simulink library "Lib_Piccolo"  (R2018b)
settings: Solver=VariableStepAuto  StartTime=0.0  StopTime=10.0  RelTol=1e-3
values from neighbouring files (symbols this model uses):
  AccelErrInt2Brakes = 0.15    [SimulationControlConfig16P.m]    (also in SimulationControlConfig16P_LEGACY.m; SimulationControlConfigTAILLESS.m = 0.2; SimulationControlConfigUTAIL.m = 0.2)
  AileronMax = 25    [SimulationControlConfig16P.m]    (also in SimulationControlConfig16P_LEGACY.m; SimulationControlConfigTAILLESS.m; SimulationControlConfigUTAIL.m)
  AileronPower = 0.00268    [SimulationControlConfig16P.m]    (also in SimulationControlConfig16P_LEGACY.m; SimulationControlConfigTAILLESS.m; SimulationControlConfigUTAIL.m)
  AileronSurfaceMax = 45    [SimulationControlConfig16P.m]    (also in SimulationControlConfig16P_LEGACY.m)
  AileronTrim = 0    [SimulationControlConfig16P.m]    (also in SimulationControlConfig16P_LEGACY.m; SimulationControlConfigTAILLESS.m; SimulationControlConfigUTAIL.m)
  Alt = 1000 + TerrainHeight    [SimulationStateConfig.m]
  AltCruise_m = testPlans(testIndx).terrainElevation * 0.3048 + 200    [SimulationControlConfig16P.m]    (also in SimulationControlConfigTAILLESS.m = 1083; SimulationControlConfigUTAIL.m = testPlans(testIndx).terrainElevation * 0.3048 + 152)
  AltitudeRate2PitchCmdIntegratorInit = 0.1    [SimulationControlPre.m]
  AltMax = 10000    [SimulationControlConfig16P.m]    (also in SimulationControlConfig16P_LEGACY.m; SimulationControlConfigTAILLESS.m; SimulationControlConfigUTAIL.m)
  AltMaxAccel = 1.25    [SimulationControlConfig16P.m]    (also in SimulationControlConfig16P_LEGACY.m = 0.9; SimulationControlConfigTAILLESS.m = 1.7; SimulationControlConfigUTAIL.m = 2)
  AltMin = 0    [SimulationControlConfig16P.m]    (also in SimulationControlConfig16P_LEGACY.m; SimulationControlConfigTAILLESS.m; SimulationControlConfigUTAIL.m)
  AltRateCmd2Pitch = 0.50    (= 0.5)    [SimulationControlConfig16P.m]    (also in SimulationControlConfig16P_LEGACY.m = 0.6; SimulationControlConfigTAILLESS.m = 0.2; SimulationControlConfigUTAIL.m = 0.3)
  AltRateError2Pitch = 0.40    (= 0.4)    [SimulationControlConfig16P.m]    (also in SimulationControlConfig16P_LEGACY.m; SimulationControlConfigTAILLESS.m = 0.55; SimulationControlConfigUTAIL.m = 0.55)
  AltRateErrorInt2Pitch = 0.50    (= 0.5)    [SimulationControlConfig16P.m]    (also in SimulationControlConfig16P_LEGACY.m = 0.45; SimulationControlConfigTAILLESS.m; SimulationControlConfigUTAIL.m = 0.75)
  AltRateLpfCutOff = 3    [SimulationControlConfig16P.m]    (also in SimulationControlConfig16P_LEGACY.m; SimulationControlConfigTAILLESS.m = 2; SimulationControlConfigUTAIL.m = 2)
  AutoNosegear2Rudder = 26    [SimulationControlConfig16P.m]    (also in SimulationControlConfig16P_LEGACY.m; SimulationControlConfigTAILLESS.m = 25.2; SimulationControlConfigUTAIL.m = 14)
  b = 5.54    [SimulationControlConfig16P.m]    (also in SimulationControlConfig16P_LEGACY.m; SimulationControlConfigTAILLESS.m = 2.37; SimulationControlConfigUTAIL.m = 2.37)
  Bank2AileronIntegratorInit = 0    [SimulationControlPre.m]
  BankMax_User = BankMax_User/180*pi    (= 0.523598775598)    [SimulationControlConfig16P.m]    (also in SimulationControlConfig16P_LEGACY.m; SimulationControlConfigTAILLESS.m = 0.610865238198; SimulationControlConfigUTAIL.m = 0.628318530718)
  baseLegFlaps = 20    [SimulationControlConfig16P.m]    (also in SimulationControlConfig16P_LEGACY.m = 0; SimulationControlConfigTAILLESS.m = 15; SimulationControlConfigUTAIL.m = 10)
  C = GeneticOpt.C    [SimulationCostFunction.m]
  c = Sw/b    (= 0.841696750903)    [SimulationControlConfig16P.m]    (also in SimulationControlConfig16P_LEGACY.m; SimulationControlConfigTAILLESS.m = 0.354008438819; SimulationControlConfigUTAIL.m = 0.354008438819)
  cell2WheelFactorMG = 5.98    [SimulationSensorConfig16P_LEGACY.m]
  cell2WheelFactorNG = 1    [SimulationSensorConfig16P_LEGACY.m]
  cellSatMaxMG = 15000    [SimulationSensorConfig16P.m]    (also in SimulationSensorConfig16P_LEGACY.m; SimulationSensorConfigTAILLESS7P.m; SimulationSensorConfigUTAIL7P.m)
  cellSatMaxNG = 1000    [SimulationSensorConfig16P.m]    (also in SimulationSensorConfig16P_LEGACY.m; SimulationSensorConfigTAILLESS7P.m; SimulationSensorConfigUTAIL7P.m)
  cellSatMinMG = -15000    [SimulationSensorConfig16P.m]    (also in SimulationSensorConfig16P_LEGACY.m; SimulationSensorConfigTAILLESS7P.m; SimulationSensorConfigUTAIL7P.m)
  cellSatMinNG = -1000    [SimulationSensorConfig16P.m]    (also in SimulationSensorConfig16P_LEGACY.m; SimulationSensorConfigTAILLESS7P.m; SimulationSensorConfigUTAIL7P.m)
  CL_Limit = CL_Max    (= 0.54)    [SimulationControlConfig16P.m]    (also in SimulationControlConfig16P_LEGACY.m; SimulationControlConfigTAILLESS.m; SimulationControlConfigUTAIL.m = 0.53)
  CL_Max = 0.54    [SimulationControlConfig16P.m]    (also in SimulationControlConfig16P_LEGACY.m; SimulationControlConfigTAILLESS.m; SimulationControlConfigUTAIL.m = 0.53)
  CL_Max_Nom = 0.465    [SimulationControlConfig16P.m]    (also in SimulationControlConfig16P_LEGACY.m; SimulationControlConfigTAILLESS.m = 0.39; SimulationControlConfigUTAIL.m)
  CL_Min = 0    [SimulationControlConfig16P.m]    (also in SimulationControlConfig16P_LEGACY.m; SimulationControlConfigTAILLESS.m; SimulationControlConfigUTAIL.m)
  ClimbMaxFraction = 0.35    [SimulationControlConfig16P.m]    (also in SimulationControlConfig16P_LEGACY.m = 0.24; SimulationControlConfigTAILLESS.m = 0.19; SimulationControlConfigUTAIL.m = 0.21)
  ClimboutMaxBank = 7.0    (= 7)    [SimulationControlConfig16P.m]    (also in SimulationControlConfig16P_LEGACY.m; SimulationControlConfigTAILLESS.m = 5; SimulationControlConfigUTAIL.m)
  ClimboutTimer = 7.0    (= 7)    [SimulationControlConfig16P.m]    (also in SimulationControlConfig16P_LEGACY.m; SimulationControlConfigTAILLESS.m; SimulationControlConfigUTAIL.m)
  dCl_per_dFlap = 0.005581818    [SimulationControlConfig16P.m]    (also in SimulationControlConfig16P_LEGACY.m = 0; SimulationControlConfigTAILLESS.m = 0; SimulationControlConfigUTAIL.m = 0)
  DecelerationCmd = 3.1    [SimulationControlConfig16P.m]    (also in SimulationControlConfig16P_LEGACY.m; SimulationControlConfigTAILLESS.m = 0.1; SimulationControlConfigUTAIL.m = 0.1)
  DeRotateLogicEndTimer = abs((NoseDownLimit_Deg-1)/DeRotateRamp_Dps)    [SimulationControlConfig16P.m]    (also in SimulationControlConfig16P_LEGACY.m; SimulationControlConfigTAILLESS.m; SimulationControlConfigUTAIL.m)
  DeRotateLogicHoldNoseUpTimer = 0.1    [SimulationControlConfig16P.m]    (also in SimulationControlConfig16P_LEGACY.m; SimulationControlConfigTAILLESS.m; SimulationControlConfigUTAIL.m)
  DeRotateLogicTimerTimeout = 2    [SimulationControlConfig16P.m]    (also in SimulationControlConfig16P_LEGACY.m; SimulationControlConfigTAILLESS.m; SimulationControlConfigUTAIL.m)
  DeRotateLowerCmdSaturation = 0    [SimulationControlConfig16P.m]    (also in SimulationControlConfig16P_LEGACY.m; SimulationControlConfigTAILLESS.m; SimulationControlConfigUTAIL.m)
  DeRotateRamp_Dps = 3    [SimulationControlConfig16P.m]    (also in SimulationControlConfig16P_LEGACY.m; SimulationControlConfigTAILLESS.m = 8; SimulationControlConfigUTAIL.m = 8)
  DeRotateUpperCmdSaturation = 7    [SimulationControlConfig16P.m]    (also in SimulationControlConfig16P_LEGACY.m; SimulationControlConfigTAILLESS.m; SimulationControlConfigUTAIL.m)
  DescentMaxFraction = 0.22    [SimulationControlConfig16P.m]    (also in SimulationControlConfig16P_LEGACY.m = 0.2; SimulationControlConfigTAILLESS.m = 0.17; SimulationControlConfigUTAIL.m = 0.17)
  DesktopSimTerrainOffset_m = 0.406    [SimulationAircraftConfig.m]
  downwindFlaps = 0    [SimulationControlConfig16P.m]    (also in SimulationControlConfig16P_LEGACY.m; SimulationControlConfigTAILLESS.m; SimulationControlConfigUTAIL.m)
  DP_init = 0.5*1.225*V_init^2    [SimulationControlConfig16P.m]    (also in SimulationControlConfig16P_LEGACY.m; SimulationControlConfigTAILLESS.m; SimulationControlConfigUTAIL.m)
  dscNoiseMG = 1    [SimulationSensorConfig16P_LEGACY.m]
  dscNoiseNG = 0.25    [SimulationSensorConfig16P_LEGACY.m]
  DSCnumBits = 24    [SimulationSensorConfig16P.m]    (also in SimulationSensorConfig16P_LEGACY.m; SimulationSensorConfigTAILLESS7P.m; SimulationSensorConfigUTAIL7P.m)
  DSCRangeMaxMG = 15000    [SimulationSensorConfig16P.m]    (also in SimulationSensorConfig16P_LEGACY.m; SimulationSensorConfigTAILLESS7P.m; SimulationSensorConfigUTAIL7P.m)
  DSCRangeMaxNG = 1000    [SimulationSensorConfig16P.m]    (also in SimulationSensorConfig16P_LEGACY.m; SimulationSensorConfigTAILLESS7P.m; SimulationSensorConfigUTAIL7P.m)
  DSCRangeMinMG = -15000    [SimulationSensorConfig16P.m]    (also in SimulationSensorConfig16P_LEGACY.m; SimulationSensorConfigTAILLESS7P.m; SimulationSensorConfigUTAIL7P.m)
  DSCRangeMinNG = -1000    [SimulationSensorConfig16P.m]    (also in SimulationSensorConfig16P_LEGACY.m; SimulationSensorConfigTAILLESS7P.m; SimulationSensorConfigUTAIL7P.m)
  dt = DLLSim.dt    [SimulationTimeStep.m]    (also in SimulationTrim.m = 0.02)
  EarlyTouchdownThreshold = 3.0    (= 3)    [SimulationControlConfig16P.m]    (also in SimulationControlConfig16P_LEGACY.m; SimulationControlConfigTAILLESS.m = 2.2; SimulationControlConfigUTAIL.m = 2.5)
  ElevatorDeflectionRate = 15    [SimulationControlConfig16P.m]    (also in SimulationControlConfig16P_LEGACY.m = 12; SimulationControlConfigTAILLESS.m = 10; SimulationControlConfigUTAIL.m = 12)
  ElevatorMax = 25    [SimulationControlConfig16P.m]    (also in SimulationControlConfig16P_LEGACY.m; SimulationControlConfigTAILLESS.m; SimulationControlConfigUTAIL.m)
  ElevatorPower = -0.002209    [SimulationControlConfig16P.m]    (also in SimulationControlConfig16P_LEGACY.m; SimulationControlConfigTAILLESS.m = -0.002956; SimulationControlConfigUTAIL.m = -0.00205983)
  ElevatorTrim = -3.5    [SimulationControlConfig16P.m]    (also in SimulationControlConfig16P_LEGACY.m; SimulationControlConfigTAILLESS.m = -6; SimulationControlConfigUTAIL.m = -8)
  elevonBias = 0    [SimulationControlConfig16P.m]    (also in SimulationControlConfig16P_LEGACY.m; SimulationControlConfigTAILLESS.m; SimulationControlConfigUTAIL.m)
  Enable_TAS_Protection = 0    [SimulationControlConfig16P.m]    (also in SimulationControlConfig16P_LEGACY.m; SimulationControlConfigTAILLESS.m; SimulationControlConfigUTAIL.m)
  EnableCrossTrackAbort = 1    [SimulationControlConfig16P.m]    (also in SimulationControlConfigTAILLESS.m; SimulationControlConfigUTAIL.m)
  EnergyBandwidth = 0.02    [SimulationControlConfig16P.m]    (also in SimulationControlConfig16P_LEGACY.m; SimulationControlConfigTAILLESS.m = 0.06; SimulationControlConfigUTAIL.m = 0.06)
  EngineLhFuelCut = 0    [SimulationAircraftConfig.m]
  EngineRhFuelCut = 0    [SimulationAircraftConfig.m]
  FastThrottleRate = 0.075    [SimulationControlConfig16P.m]    (also in SimulationControlConfig16P_LEGACY.m = 0.05; SimulationControlConfigTAILLESS.m = 0.1; SimulationControlConfigUTAIL.m = 0.1)
  FilterWarmUpTime = 2    [SimulationSensorConfig16P.m]    (also in SimulationSensorConfig16P_LEGACY.m; SimulationSensorConfigTAILLESS7P.m; SimulationSensorConfigUTAIL7P.m)
  finalApproachFlaps = 20    [SimulationControlConfig16P.m]    (also in SimulationControlConfig16P_LEGACY.m = 0; SimulationControlConfigTAILLESS.m = 22; SimulationControlConfigUTAIL.m = 10)
  FinalDescentSlope_Deg = testPlans(testIndx).descentSlope    [SimulationControlConfig16P.m]    (also in SimulationControlConfig16P_LEGACY.m; SimulationControlConfigTAILLESS.m; SimulationControlConfigUTAIL.m)
  flapMax = 0    [SimulationControlConfig16P.m]    (also in SimulationControlConfig16P_LEGACY.m; SimulationControlConfigTAILLESS.m; SimulationControlConfigUTAIL.m)
  flapRate = 7.5    [SimulationControlConfig16P.m]    (also in SimulationControlConfig16P_LEGACY.m; SimulationControlConfigTAILLESS.m = 6.6; SimulationControlConfigUTAIL.m)
  FlareHeight = 5    [SimulationControlConfig16P.m]    (also in SimulationControlConfig16P_LEGACY.m = 4.8; SimulationControlConfigTAILLESS.m = 2.5; SimulationControlConfigUTAIL.m = 2)
  FlareVerticalRate_mps = -0.4    [SimulationControlConfig16P.m]    (also in SimulationControlConfig16P_LEGACY.m = -0.5; SimulationControlConfigTAILLESS.m = -0.15; SimulationControlConfigUTAIL.m = -0.15)
  Fp_Aileron = 0.55*2*pi*RollRateLpfCutoff*dt    [SimulationControlConfig16P.m]    (also in SimulationControlConfig16P_LEGACY.m; SimulationControlConfigTAILLESS.m; SimulationControlConfigUTAIL.m)
  Fp_Alt = 0.55*AltBandwidth    (= 0.099)    [SimulationControlConfig16P.m]    (also in SimulationControlConfig16P_LEGACY.m; SimulationControlConfigTAILLESS.m = 0.587477826221; SimulationControlConfigUTAIL.m = 0.69115038379)
  Fp_AltRate = 0.55*2*pi*AltRateLpfCutOff*dt    [SimulationControlConfig16P.m]    (also in SimulationControlConfig16P_LEGACY.m; SimulationControlConfigTAILLESS.m; SimulationControlConfigUTAIL.m)
  Fp_Elevator = 0.55*2*pi*PitchRateLpfCutoff*dt    [SimulationControlConfig16P.m]    (also in SimulationControlConfig16P_LEGACY.m; SimulationControlConfigTAILLESS.m; SimulationControlConfigUTAIL.m)
  Fp_Energy = 0.55*2*pi*EnergyBandwidth    (= 0.069115038379)    [SimulationControlConfig16P.m]    (also in SimulationControlConfig16P_LEGACY.m; SimulationControlConfigTAILLESS.m = 0.207345115137; SimulationControlConfigUTAIL.m = 0.207345115137)
  Fp_Energy2 = 0.55*2*pi*EnergyBandwidth*dt    [SimulationControlConfig16P.m]    (also in SimulationControlConfig16P_LEGACY.m; SimulationControlConfigTAILLESS.m; SimulationControlConfigUTAIL.m)
  Fp_Pitch = 0.55*2*pi*PitchBandwidth    (= 2.76460153516)    [SimulationControlConfig16P.m]    (also in SimulationControlConfig16P_LEGACY.m = 3.11017672705; SimulationControlConfigTAILLESS.m = 3.80132711084; SimulationControlConfigUTAIL.m = 2.41902634326)
  Fp_Pitch_2 = 0.55*2*pi*PitchBandwidth*dt    [SimulationControlConfig16P.m]    (also in SimulationControlConfig16P_LEGACY.m; SimulationControlConfigTAILLESS.m; SimulationControlConfigUTAIL.m)
  Fp_Roll = RollBandwidth^2    (= 1)    [SimulationControlConfig16P.m]    (also in SimulationControlConfig16P_LEGACY.m = 1.44; SimulationControlConfigTAILLESS.m; SimulationControlConfigUTAIL.m)
  Fp_Rudder = 0.55*2*pi*YawRateLpfCutoff*dt    [SimulationControlConfig16P.m]    (also in SimulationControlConfig16P_LEGACY.m; SimulationControlConfigTAILLESS.m; SimulationControlConfigUTAIL.m)
  Fp_TAS = 0.55*2*pi*TASBandwidth    (= 0.103672557568)    [SimulationControlConfig16P.m]    (also in SimulationControlConfig16P_LEGACY.m; SimulationControlConfigTAILLESS.m = 0.172787595947; SimulationControlConfigUTAIL.m = 0.172787595947)
  Fp_TAS_Filter = 2*pi*TasLpfCutoff*dt    [SimulationControlConfig16P.m]    (also in SimulationControlConfig16P_LEGACY.m; SimulationControlConfigTAILLESS.m; SimulationControlConfigUTAIL.m)
  Fp_Turn = 0.55*2*pi*TurnErrLPFcutoff    (= 0.0345575191895)    [SimulationControlConfig16P.m]    (also in SimulationControlConfig16P_LEGACY.m; SimulationControlConfigTAILLESS.m = 0.172787595947; SimulationControlConfigUTAIL.m = 0.172787595947)
  Fp_TurnDerr = 0.55*2*pi*TurnDerivativeLPFcutoff    (= 0.0345575191895)    [SimulationControlConfig16P.m]    (also in SimulationControlConfig16P_LEGACY.m; SimulationControlConfigTAILLESS.m = 0.172787595947; SimulationControlConfigUTAIL.m = 0.172787595947)
  FTV = 3    [SimulationAircraftConfig.m]
  ftvStaticPositionError = 1/1.18    (= 0.847457627119)    [SimulationSensorConfig16P.m]    (also in SimulationSensorConfig16P_LEGACY.m; SimulationSensorConfigTAILLESS7P.m = 1; SimulationSensorConfigUTAIL7P.m = 1)
  g = 9.81    [SimulationStateConfig.m]
  GustSpd_Kts = testPlans(testIndx).gustSpd    [SimulationStateConfig.m]
  GustTriggerVal = testPlans(testIndx).gustTriggerVal    [SimulationStateConfig.m]
  HeadingErr2TurnRate = 0.5    [SimulationControlConfig16P.m]    (also in SimulationControlConfig16P_LEGACY.m; SimulationControlConfigTAILLESS.m; SimulationControlConfigUTAIL.m)
  HeadingErrDer2TurnRate = 0.3    [SimulationControlConfig16P.m]    (also in SimulationControlConfig16P_LEGACY.m; SimulationControlConfigTAILLESS.m; SimulationControlConfigUTAIL.m)
  IASbounce = IASstall*0.8    [SimulationControlPre.m]
  IAScruiseCMD = sqrt(2*m*9.81/(1.225*Sw*CL_cruise))    [SimulationControlConfig16P.m]    (also in SimulationControlConfig16P_LEGACY.m; SimulationControlConfigTAILLESS.m; SimulationControlConfigUTAIL.m)
  IASfinalCMD = 1.12 * IASmin    [SimulationControlConfig16P.m]    (also in SimulationControlConfig16P_LEGACY.m = 1.10 * IASmin; SimulationControlConfigTAILLESS.m = 1.10 * IASmin; SimulationControlConfigUTAIL.m = 1.15 * IASmin)
  IASflareCMD = IASstall    [SimulationControlConfig16P.m]    (also in SimulationControlConfig16P_LEGACY.m; SimulationControlConfigTAILLESS.m; SimulationControlConfigUTAIL.m)
  IASmax = 64    [SimulationControlConfig16P.m]    (also in SimulationControlConfig16P_LEGACY.m = 46; SimulationControlConfigTAILLESS.m = 38.58; SimulationControlConfigUTAIL.m = 35)
  IASmin = sqrt(2*m*9.81/(1.225*Sw*0.9*CL_Max_Nom))    [SimulationControlConfig16P.m]    (also in SimulationControlConfig16P_LEGACY.m; SimulationControlConfigTAILLESS.m; SimulationControlConfigUTAIL.m)
  IASshortCMD = IASstall    [SimulationControlConfig16P.m]    (also in SimulationControlConfig16P_LEGACY.m; SimulationControlConfigTAILLESS.m; SimulationControlConfigUTAIL.m)
  IASstall = sqrt(2*m*9.81/(1.225*Sw*CL_Max))    [SimulationControlConfig16P.m]    (also in SimulationControlConfig16P_LEGACY.m; SimulationControlConfigTAILLESS.m; SimulationControlConfigUTAIL.m)
  inFlight = 1    [SimulationControlConfig16P.m]    (also in SimulationControlConfigTAILLESS.m; SimulationControlConfigUTAIL.m)
  JetCatOffset = 5    [SimulationControlConfig16P.m]    (also in SimulationControlConfig16P_LEGACY.m)
  LaunchRollingElevator = -1.5    [SimulationControlConfig16P.m]    (also in SimulationControlConfig16P_LEGACY.m; SimulationControlConfigTAILLESS.m = 1; SimulationControlConfigUTAIL.m = 1)
  ldg_NosegearMax = 10    [SimulationControlConfig16P.m]    (also in SimulationControlConfig16P_LEGACY.m; SimulationControlConfigTAILLESS.m; SimulationControlConfigUTAIL.m)
  ldg_TrackVyErrInt2Nosegear = 0.1250    (= 0.125)    [SimulationControlConfig16P.m]    (also in SimulationControlConfig16P_LEGACY.m; SimulationControlConfigTAILLESS.m = 0.00714285714286; SimulationControlConfigUTAIL.m = 0.00714285714286)
  ldg_TrackVyErrPro2Nosegear = 0.35    [SimulationControlConfig16P.m]    (also in SimulationControlConfig16P_LEGACY.m; SimulationControlConfigTAILLESS.m = 0.0546666666667; SimulationControlConfigUTAIL.m = 0.0546666666667)
  ldg_TrackY2Vy = 0.07    [SimulationControlConfig16P.m]    (also in SimulationControlConfig16P_LEGACY.m; SimulationControlConfigTAILLESS.m = 0.17; SimulationControlConfigUTAIL.m = 0.17)
  ldg_Vy2NosegearScalingPower = 1.075    [SimulationControlConfig16P.m]    (also in SimulationControlConfig16P_LEGACY.m; SimulationControlConfigTAILLESS.m = 0.6; SimulationControlConfigUTAIL.m = 0.5)
  ldg_Y2VyScalingPower = 0.175    [SimulationControlConfig16P.m]    (also in SimulationControlConfig16P_LEGACY.m; SimulationControlConfigTAILLESS.m = 0; SimulationControlConfigUTAIL.m = 0)
  ldg_YawRate2Nosegear = 0.175    [SimulationControlConfig16P.m]    (also in SimulationControlConfig16P_LEGACY.m; SimulationControlConfigTAILLESS.m = 0.065; SimulationControlConfigUTAIL.m = 0.065)
  LiftSlope = 0.064285    [SimulationControlConfig16P.m]    (also in SimulationControlConfig16P_LEGACY.m; SimulationControlConfigTAILLESS.m = 0.058631; SimulationControlConfigUTAIL.m)
  LPFaileronInit = 0    [SimulationControlPre.m]
  LPFclestInit = 0    [SimulationControlPre.m]
  LPFenergyFFInit = 0    [SimulationControlPre.m]
  LPFtasInit = V_init + 2    [SimulationControlPre.m]
  LPFthrottleInit = ThrottleTrim    [SimulationControlPre.m]
  LPFturnErrInit = 0    [SimulationControlPre.m]
  ... (+115 more)
undefined symbols (not defined in the file or in its folder): abortFlag, alphaHPF, apmDelay, BRWNOUT, CRAWOR, CRAWUR, DiscIntNeverNeededParam, DLLSim, DLLSimStep, ECOMOR, ECOMUR, Fp_Tas, GustTrigger_HeightAgl_m, IPSTAT, LCINTEG, Ldg_Persist_Time, LOWER_FLAGS, MSG_ENABLE, NoiseStd, OLDVAL, OVERRIDE_ENABLE, OVERRIDE_VALUE, REBOOT, reversionEnable, revIASMax, revIASMin, revPitchMax, revPitchMin, revPitchRateMax, revRollMax, revRollRateMax, SAMPLE, SCALON, SensorModel, sigbuilder_block, Sim_Vx, Sim_Vy, Sim_Vz, Sim_Xpos, Sim_Ypos, Sim_Zpos, SYSOR, SYSUR, TARE, TEMPOR, TEMPUR, testIndx, testPlan, testPlans, Trim_piccoloInCmd, Trim_REFSI_FD_IN_nmodeCgShifterCmd_Ft, Trim_REFSI_FD_IN_nmodeFlapLhIBCmd_Deg, Trim_REFSI_FD_IN_nmodeFlapLhOBCmd_Deg, Trim_REFSI_FD_IN_nmodeFlapRhIBCmd_Deg, Trim_REFSI_FD_IN_nmodeFlapRhOBCmd_Deg, Trim_REFSI_FD_IN_nmodeSlatLhCmd_Deg, Trim_REFSI_FD_IN_nmodeSlatRhCmd_Deg, Trim_REFSI_FD_IN_nmodeSplrLhInbdCmd_Deg, Trim_REFSI_FD_IN_nmodeSplrLhOutbdCmd_Deg ... (+5)
libraries: simulink x866, aerolibconvert2 x60, $bdroot x52, aerolibatmos2 x5, dspswit3 x5, simulink_extras x4, dsparch4 x2, Lib_Piccolo_Alt x2, eeGeneralControl x1, dspindex x1
(part 10 of 44)

== system Lib_Piccolo/Control Allocation/M2 ==
  note: For 16.5% U-tail:
      | Aileron: aileron, inboard elevon, outboard elevon
      | Elevator: aft-flap, U-tail elevator,
      | Rudder: pylon rudder, winglet rudder, U-tail rudder
      |
      | For 16.5% Tailless (w/o U-tail elevator and U-tail rudder):
      | Aileron: aileron, inboard elevon, outboard elevon
      | Elevator: aft-flap, inboard elvon, outboard elevon
      | Rudder: pylon rudder, winglet rudder
  Aileron : Inport
  Elevator : Inport  Port=2
  Rudder : Inport  Port=3
  Throttle : Inport  Port=4
  Nosegear : Inport  Port=5
  Brake : Inport  Port=6
  Flap : Inport  Port=7
  Feedback Bus : Inport  Port=8
  Bus Creator : BusCreator  Inputs=10
  Bus Creator1 : BusCreator  Inputs=4
  Bus Creator2 : BusCreator  Inputs=2
  Bus Creator3 : BusCreator  Inputs=2
  Bus Creator4 : BusCreator  Inputs=2
  Constant : Constant  Value=FTV
  Constant1 : Constant  Value=0
  Constant2 : Constant  Value=elevonBias
  Gain{1..5,8..9,12,14,16..17} (11 alike) : Gain
  Gain{10..11,13,15} (4 alike) : Gain  Gain=-1
  Signal Specification : SignalSpecification  Dimensions=[1 1]  SampleTime=dt
  Signal Specification1 : SignalSpecification  Dimensions=[1 1]  SampleTime=dt
  Signal Specification2 : SignalSpecification  Dimensions=[1 1]  SampleTime=dt
  SlatLhPosnDeg : Constant  Value=Trim_REFSI_FD_IN_nmodeSlatLhCmd_Deg
  StabCmdDeg : Constant  Value=Trim_REFSI_FD_IN_nmodeStabCmd
  Surface Mixing Function : MATLAB Function  TreatAsAtomicUnit=on
  Switch : Switch  Criteria=u2 > Threshold  Threshold=2
  Terminator : Terminator
  Variant Model : $bdroot/Control Allocation/M2 Flap-to-Drag /Variant Model  SystemSampleTime=-1
  nmodeTlaLhCmdDeg3 : Constant  Value=Trim_REFSI_FD_IN_nmodeSplrLhOutbdCmd_Deg
  "Aileron_Deg " : Outport
  "InboardElevon_Deg " : Outport  Port=2
  OutboardElevon_Deg : Outport  Port=3
  "U-TailElevator_Deg " : Outport  Port=4
  Aft-Flap_Deg : Outport  Port=5
  PylonRudder_Deg : Outport  Port=6
  WingletRudder_Deg : Outport  Port=7
  U-tailRudder_Deg : Outport  Port=8
  "Throttle_Pct " : Outport  Port=9
  Nosegear_Deg : Outport  Port=10
  Brake (0-1) : Outport  Port=11
  Flaps_Deg : Outport  Port=12
  Slats_Deg : Outport  Port=13
  Spoilers_Deg : Outport  Port=14
  Stabilizer_Deg : Outport  Port=15
  tag scope: Sim_Surface=global
  wires:
  Elevator/1 -> Bus Creator/2, Signal Specification1/1  "Sim_ElevatorCmd"
  Aileron/1 -> Bus Creator/1, Signal Specification/1  "Sim_AileronCmd"
  Rudder/1 -> Bus Creator/3, Signal Specification2/1  "Sim_RudderCmd"
  Nosegear/1 -> Bus Creator/5, Nosegear_Deg/1  "Sim_NosegearCmd"
  Brake/1 -> Brake (0-1)/1, Bus Creator/6  "Sim_BrakeCmd"
  Bus Creator/1 -> [Sim_Surface]
  Throttle/1 -> Variant Model/1, Bus Creator/4  "Sim_ThrottleCmd"
  Variant Model/1 -> Gain16/1, Gain17/1  "Sim_ThrottleCmd"
  Bus Creator1/1 -> "Aileron_Deg "/1
  Bus Creator2/1 -> "InboardElevon_Deg "/1
  Bus Creator3/1 -> OutboardElevon_Deg/1
  Gain8/1 -> Bus Creator1/1  "PrtAileronUpperCmd_Deg"
  Gain9/1 -> Bus Creator1/2  "PrtAileronLowerCmd_Deg"
  Gain10/1 -> Bus Creator1/3  "StbdAileronUpperCmd_Deg"
  Gain11/1 -> Bus Creator1/4  "StbdAileronLowerCmd_Deg"
  Gain12/1 -> Bus Creator2/1  "PrtInbElevonCmd_Deg"
  Gain13/1 -> Bus Creator2/2  "StbdInbElevonCmd_Deg"
  Gain14/1 -> Bus Creator3/1  "PrtOutElevonCmd_Deg"
  Gain15/1 -> Bus Creator3/2  "StbdOutElevonCmd_Deg"
  Gain16/1 -> Bus Creator4/1  "PrtThrottleCmd_Pct"
  Bus Creator4/1 -> "Throttle_Pct "/1
  Gain17/1 -> Bus Creator4/2  "StbdThrottleCmd_Pct"
  SlatLhPosnDeg/1 -> Bus Creator/8, Slats_Deg/1  "Sim_SlatsCmd"
  nmodeTlaLhCmdDeg3/1 -> Bus Creator/9, Spoilers_Deg/1  "Sim_SpoilersCmd"
  Feedback Bus/1 -> Terminator/1
  StabCmdDeg/1 -> Bus Creator/10, Stabilizer_Deg/1  "Sim_StabilizerCmd"
  Flap/1 -> Surface Mixing Function/4(Pic_FlapCmd), Bus Creator/7, Flaps_Deg/1  "Sim_FlapsCmd"
  Surface Mixing Function/1(PrtAileronUpperCmd) -> Gain8/1
  Surface Mixing Function/2(PrtAileronLowerCmd) -> Gain9/1
  Surface Mixing Function/3(StbdAileronUpperCmd) -> Gain10/1
  Surface Mixing Function/4(StbdAileronLowerCmd) -> Gain11/1
  Surface Mixing Function/13(UTailRudderCmd) -> Gain5/1
  Surface Mixing Function/12(WingletRudderCmd) -> Gain4/1
  Surface Mixing Function/11(PylonRudderCmd) -> Gain3/1
  Surface Mixing Function/10(AftFlapCmd) -> Gain2/1
  Surface Mixing Function/9(ElevatorUtailCmd) -> Gain1/1
  Surface Mixing Function/8(StbdOutdElevonCmd) -> Gain15/1
  Surface Mixing Function/7(PrtOutElevonCmd) -> Gain14/1
  Surface Mixing Function/6(StbdInbdElevonCmd) -> Gain13/1
  Surface Mixing Function/5(PrtInbElevonCmd) -> Gain12/1
  Gain1/1 -> "U-TailElevator_Deg "/1  "UtailElevator_Deg"
  Gain2/1 -> Aft-Flap_Deg/1  "AftFlap_deg"
  Gain3/1 -> PylonRudder_Deg/1  "PylonRudder_Deg"
  Gain5/1 -> U-tailRudder_Deg/1  "UtailRudder_Deg"
  Signal Specification/1 -> Surface Mixing Function/1(Pic_AileronCmd)
  Signal Specification2/1 -> Surface Mixing Function/3(Pic_RudderCmd)
  Signal Specification1/1 -> Surface Mixing Function/2(Pic_ElevatorCmd)
  Constant/1 -> Switch/2
  Switch/1 -> WingletRudder_Deg/1  "WingletRudder_Deg"
  Constant1/1 -> Switch/3
  Gain4/1 -> Switch/1
  Constant2/1 -> Surface Mixing Function/5(elevonBias)

== system Lib_Piccolo/Control Allocation/M2 Flap-to-Drag  ==
  note: For 16.5% U-tail:
      | Aileron: aileron, inboard elevon, outboard elevon
      | Elevator: aft-flap, U-tail elevator,
      | Rudder: pylon rudder, winglet rudder, U-tail rudder
      |
      | For 16.5% Tailless (w/o U-tail elevator and U-tail rudder):
      | Aileron: aileron, inboard elevon, outboard elevon
      | Elevator: aft-flap, inboard elvon, outboard elevon
      | Rudder: pylon rudder, winglet rudder
  Aileron : Inport
  Elevator : Inport  Port=2
  Rudder : Inport  Port=3
  Throttle : Inport  Port=4
  Nosegear : Inport  Port=5
  Brake : Inport  Port=6
  Flap : Inport  Port=7
  Feedback Bus : Inport  Port=8
  Bus Creator : BusCreator  Inputs=10
  Bus Creator1 : BusCreator  Inputs=4
  Bus Creator2 : BusCreator  Inputs=2
  Bus Creator3 : BusCreator  Inputs=2
  Bus Creator4 : BusCreator  Inputs=2
  Constant : Constant  Value=FTV
  Constant1 : Constant  Value=0
  Constant2 : Constant  Value=elevonBias
  Constant3 : Constant  Value=AileronSurfaceMax
  FlapLhIBCmdDeg : Constant  Commented=on  Value=Trim_REFSI_FD_IN_nmodeFlapLhIBCmd_Deg
  FlapLhIBCmdDeg1 : Constant  Value=Trim_REFSI_FD_IN_nmodeFlapLhIBCmd_Deg
  Gain{1..5,8..9,12,14,16..17} (11 alike) : Gain
  Gain{10..11,13,15} (4 alike) : Gain  Gain=-1
  Signal Specification{,1..3} (4 alike) : SignalSpecification  Dimensions=[1 1]  SampleTime=dt
  SlatLhPosnDeg : Constant  Value=Trim_REFSI_FD_IN_nmodeSlatLhCmd_Deg
  StabCmdDeg : Constant  Value=Trim_REFSI_FD_IN_nmodeStabCmd
  Surface Mixing Function : MATLAB Function  TreatAsAtomicUnit=on
  Switch : Switch  Criteria=u2 > Threshold  Threshold=2
  Terminator : Terminator
  Variant Model : Subsystem  Variant=on
  nmodeTlaLhCmdDeg3 : Constant  Value=Trim_REFSI_FD_IN_nmodeSplrLhOutbdCmd_Deg
  "Aileron_Deg " : Outport
  "InboardElevon_Deg " : Outport  Port=2
  OutboardElevon_Deg : Outport  Port=3
  "U-TailElevator_Deg " : Outport  Port=4
  Aft-Flap_Deg : Outport  Port=5
  PylonRudder_Deg : Outport  Port=6
  WingletRudder_Deg : Outport  Port=7
  U-tailRudder_Deg : Outport  Port=8
  "Throttle_Pct " : Outport  Port=9
  Nosegear_Deg : Outport  Port=10
  Brake (0-1) : Outport  Port=11
  Flaps_Deg : Outport  Port=12
  Slats_Deg : Outport  Port=13
  Spoilers_Deg : Outport  Port=14
  Stabilizer_Deg : Outport  Port=15
  tag scope: Sim_Surface=global
  wires:
  Gain4/1 -> Switch/1
  Constant1/1 -> Switch/3
  Switch/1 -> WingletRudder_Deg/1  "WingletRudder_Deg"
  Constant/1 -> Switch/2
  Signal Specification1/1 -> Surface Mixing Function/2(Pic_ElevatorCmd)
  Signal Specification2/1 -> Surface Mixing Function/3(Pic_RudderCmd)
  Signal Specification/1 -> Surface Mixing Function/1(Pic_AileronCmd)
  Gain5/1 -> U-tailRudder_Deg/1  "UtailRudder_Deg"
  Gain3/1 -> PylonRudder_Deg/1  "PylonRudder_Deg"
  Gain2/1 -> Aft-Flap_Deg/1  "AftFlap_deg"
  Gain1/1 -> "U-TailElevator_Deg "/1  "UtailElevator_Deg"
  Surface Mixing Function/5(PrtInbElevonCmd) -> Gain12/1
  Surface Mixing Function/6(StbdInbdElevonCmd) -> Gain13/1
  Surface Mixing Function/7(PrtOutElevonCmd) -> Gain14/1
  Surface Mixing Function/8(StbdOutdElevonCmd) -> Gain15/1
  Surface Mixing Function/9(ElevatorUtailCmd) -> Gain1/1
  Surface Mixing Function/10(AftFlapCmd) -> Gain2/1
  Surface Mixing Function/11(PylonRudderCmd) -> Gain3/1
  Surface Mixing Function/12(WingletRudderCmd) -> Gain4/1
  Surface Mixing Function/13(UTailRudderCmd) -> Gain5/1
  Surface Mixing Function/4(StbdAileronLowerCmd) -> Gain11/1
  Surface Mixing Function/3(StbdAileronUpperCmd) -> Gain10/1
  Surface Mixing Function/2(PrtAileronLowerCmd) -> Gain9/1
  Surface Mixing Function/1(PrtAileronUpperCmd) -> Gain8/1
  Flap/1 -> Signal Specification3/1, Bus Creator/7  "Sim_FlapsCmd"
  StabCmdDeg/1 -> Stabilizer_Deg/1, Bus Creator/10  "Sim_StabilizerCmd"
  Feedback Bus/1 -> Terminator/1
  nmodeTlaLhCmdDeg3/1 -> Spoilers_Deg/1, Bus Creator/9  "Sim_SpoilersCmd"
  SlatLhPosnDeg/1 -> Slats_Deg/1, Bus Creator/8  "Sim_SlatsCmd"
  Gain17/1 -> Bus Creator4/2  "StbdThrottleCmd_Pct"
  Bus Creator4/1 -> "Throttle_Pct "/1
  Gain16/1 -> Bus Creator4/1  "PrtThrottleCmd_Pct"
  Gain15/1 -> Bus Creator3/2  "StbdOutElevonCmd_Deg"
  Gain14/1 -> Bus Creator3/1  "PrtOutElevonCmd_Deg"
  Gain13/1 -> Bus Creator2/2  "StbdInbElevonCmd_Deg"
  Gain12/1 -> Bus Creator2/1  "PrtInbElevonCmd_Deg"
  Gain11/1 -> Bus Creator1/4  "StbdAileronLowerCmd_Deg"
  Gain10/1 -> Bus Creator1/3  "StbdAileronUpperCmd_Deg"
  Gain9/1 -> Bus Creator1/2  "PrtAileronLowerCmd_Deg"
  Gain8/1 -> Bus Creator1/1  "PrtAileronUpperCmd_Deg"
  Bus Creator3/1 -> OutboardElevon_Deg/1
  Bus Creator2/1 -> "InboardElevon_Deg "/1
  Bus Creator1/1 -> "Aileron_Deg "/1
  Variant Model/1(ThrottleCmdOut) -> Gain16/1, Gain17/1  "Sim_ThrottleCmd"
  Throttle/1 -> Variant Model/1(Sim_ThrottleCmd), Bus Creator/4  "Sim_ThrottleCmd"
  Bus Creator/1 -> [Sim_Surface]
  Brake/1 -> Bus Creator/6, Brake (0-1)/1  "Sim_BrakeCmd"
  Nosegear/1 -> Nosegear_Deg/1, Bus Creator/5  "Sim_NosegearCmd"
  Rudder/1 -> Signal Specification2/1, Bus Creator/3  "Sim_RudderCmd"
  Aileron/1 -> Signal Specification/1, Bus Creator/1  "Sim_AileronCmd"
  Elevator/1 -> Signal Specification1/1, Bus Creator/2  "Sim_ElevatorCmd"
  FlapLhIBCmdDeg1/1 -> Flaps_Deg/1  "REFSI_FD_IN_nmodeFlapLhOBPosn_Deg"
  Signal Specification3/1 -> Surface Mixing Function/4(Pic_FlapCmd)
  Constant2/1 -> Surface Mixing Function/5(elevonBias)
  Constant3/1 -> Surface Mixing Function/6(AileronMax)

== system Lib_Piccolo/Control Allocation/M2 Flaperon ==
  note: For 16.5% U-tail:
      | Aileron: aileron, inboard elevon, outboard elevon
      | Elevator: aft-flap, U-tail elevator,
      | Rudder: pylon rudder, winglet rudder, U-tail rudder
      |
      | For 16.5% Tailless (w/o U-tail elevator and U-tail rudder):
      | Aileron: aileron, inboard elevon, outboard elevon
      | Elevator: aft-flap, inboard elvon, outboard elevon
      | Rudder: pylon rudder, winglet rudder
  Aileron : Inport
  Elevator : Inport  Port=2
  Rudder : Inport  Port=3
  Throttle : Inport  Port=4
  Nosegear : Inport  Port=5
  Brake : Inport  Port=6
  Flap : Inport  Port=7
  Feedback Bus : Inport  Port=8
  Bus Creator : BusCreator  Inputs=10
  Bus Creator1 : BusCreator  Inputs=4
  Bus Creator2 : BusCreator  Inputs=2
  Bus Creator3 : BusCreator  Inputs=2
  Bus Creator4 : BusCreator  Inputs=2
  Constant : Constant  Value=FTV
  Constant1 : Constant  Value=0
  FlapLhIBCmdDeg : Constant  Commented=on  Value=Trim_REFSI_FD_IN_nmodeFlapLhIBCmd_Deg
  FlapLhIBCmdDeg1 : Constant  Value=Trim_REFSI_FD_IN_nmodeFlapLhIBCmd_Deg
  Gain{1..5,8..9,12..17} (13 alike) : Gain
  Gain10 : Gain  Gain=-1
  Gain11 : Gain  Gain=-1
  Signal Specification{,1..3} (4 alike) : SignalSpecification  Dimensions=[1 1]  SampleTime=dt
  SlatLhPosnDeg : Constant  Value=Trim_REFSI_FD_IN_nmodeSlatLhCmd_Deg
  StabCmdDeg : Constant  Value=Trim_REFSI_FD_IN_nmodeStabCmd
  Surface Mixing Function : MATLAB Function  TreatAsAtomicUnit=on
  Switch : Switch  Criteria=u2 > Threshold  Threshold=2
  Terminator : Terminator
  Variant Model : $bdroot/Control Allocation/M2 Flap-to-Drag /Variant Model  SystemSampleTime=-1  Latency=0  AutoFrameSizeCalculation=off
  nmodeTlaLhCmdDeg3 : Constant  Value=Trim_REFSI_FD_IN_nmodeSplrLhOutbdCmd_Deg
  "Aileron_Deg " : Outport
  "InboardElevon_Deg " : Outport  Port=2
  OutboardElevon_Deg : Outport  Port=3
  "U-TailElevator_Deg " : Outport  Port=4
  Aft-Flap_Deg : Outport  Port=5
  PylonRudder_Deg : Outport  Port=6
  WingletRudder_Deg : Outport  Port=7
  U-tailRudder_Deg : Outport  Port=8
  "Throttle_Pct " : Outport  Port=9
  Nosegear_Deg : Outport  Port=10
  Brake (0-1) : Outport  Port=11
  Flaps_Deg : Outport  Port=12
  Slats_Deg : Outport  Port=13
  Spoilers_Deg : Outport  Port=14
  Stabilizer_Deg : Outport  Port=15
  tag scope: Sim_Surface=global
  wires:
  Gain4/1 -> Switch/1
  Constant1/1 -> Switch/3
  Switch/1 -> WingletRudder_Deg/1  "WingletRudder_Deg"
  Constant/1 -> Switch/2
  Signal Specification1/1 -> Surface Mixing Function/2(Pic_ElevatorCmd)
  Signal Specification2/1 -> Surface Mixing Function/3(Pic_RudderCmd)
  Signal Specification/1 -> Surface Mixing Function/1(Pic_AileronCmd)
  Gain5/1 -> U-tailRudder_Deg/1  "UtailRudder_Deg"
  Gain3/1 -> PylonRudder_Deg/1  "PylonRudder_Deg"
  Gain2/1 -> Aft-Flap_Deg/1  "AftFlap_deg"
  Gain1/1 -> "U-TailElevator_Deg "/1  "UtailElevator_Deg"
  Surface Mixing Function/5(PrtInbElevonCmd) -> Gain12/1
  Surface Mixing Function/6(StbdInbdElevonCmd) -> Gain13/1
  Surface Mixing Function/7(PrtOutElevonCmd) -> Gain14/1
  Surface Mixing Function/8(StbdOutdElevonCmd) -> Gain15/1
  Surface Mixing Function/9(ElevatorUtailCmd) -> Gain1/1
  Surface Mixing Function/10(AftFlapCmd) -> Gain2/1
  Surface Mixing Function/11(PylonRudderCmd) -> Gain3/1
  Surface Mixing Function/12(WingletRudderCmd) -> Gain4/1
  Surface Mixing Function/13(UTailRudderCmd) -> Gain5/1
  Surface Mixing Function/4(StbdAileronLowerCmd) -> Gain11/1
  Surface Mixing Function/3(StbdAileronUpperCmd) -> Gain10/1
  Surface Mixing Function/2(PrtAileronLowerCmd) -> Gain9/1
  Surface Mixing Function/1(PrtAileronUpperCmd) -> Gain8/1
  Flap/1 -> Signal Specification3/1, Bus Creator/7  "Sim_FlapsCmd"
  StabCmdDeg/1 -> Stabilizer_Deg/1, Bus Creator/10  "Sim_StabilizerCmd"
  Feedback Bus/1 -> Terminator/1
  nmodeTlaLhCmdDeg3/1 -> Spoilers_Deg/1, Bus Creator/9  "Sim_SpoilersCmd"
  SlatLhPosnDeg/1 -> Slats_Deg/1, Bus Creator/8  "Sim_SlatsCmd"
  Gain17/1 -> Bus Creator4/2  "StbdThrottleCmd_Pct"
  Bus Creator4/1 -> "Throttle_Pct "/1
  Gain16/1 -> Bus Creator4/1  "PrtThrottleCmd_Pct"
  Gain15/1 -> Bus Creator3/2  "StbdOutElevonCmd_Deg"
  Gain14/1 -> Bus Creator3/1  "PrtOutElevonCmd_Deg"
  Gain13/1 -> Bus Creator2/2  "StbdInbElevonCmd_Deg"
  Gain12/1 -> Bus Creator2/1  "PrtInbElevonCmd_Deg"
  Gain11/1 -> Bus Creator1/4  "StbdAileronLowerCmd_Deg"
  Gain10/1 -> Bus Creator1/3  "StbdAileronUpperCmd_Deg"
  Gain9/1 -> Bus Creator1/2  "PrtAileronLowerCmd_Deg"
  Gain8/1 -> Bus Creator1/1  "PrtAileronUpperCmd_Deg"
  Bus Creator3/1 -> OutboardElevon_Deg/1
  Bus Creator2/1 -> "InboardElevon_Deg "/1
  Bus Creator1/1 -> "Aileron_Deg "/1
  Variant Model/1 -> Gain16/1, Gain17/1  "Sim_ThrottleCmd"
  Throttle/1 -> Variant Model/1, Bus Creator/4  "Sim_ThrottleCmd"
  Bus Creator/1 -> [Sim_Surface]
  Brake/1 -> Bus Creator/6, Brake (0-1)/1  "Sim_BrakeCmd"
  Nosegear/1 -> Nosegear_Deg/1, Bus Creator/5  "Sim_NosegearCmd"
  Rudder/1 -> Signal Specification2/1, Bus Creator/3  "Sim_RudderCmd"
  Aileron/1 -> Signal Specification/1, Bus Creator/1  "Sim_AileronCmd"
  Elevator/1 -> Signal Specification1/1, Bus Creator/2  "Sim_ElevatorCmd"
  FlapLhIBCmdDeg1/1 -> Flaps_Deg/1  "REFSI_FD_IN_nmodeFlapLhOBPosn_Deg"
  Signal Specification3/1 -> Surface Mixing Function/4(Pic_FlapCmd)

== system Lib_Piccolo/Control Allocation/M2 Flaperon and FTD ==
  note: For 16.5% U-tail:
      | Aileron: aileron, inboard elevon, outboard elevon
      | Elevator: aft-flap, U-tail elevator,
      | Rudder: pylon rudder, winglet rudder, U-tail rudder
      |
      | For 16.5% Tailless (w/o U-tail elevator and U-tail rudder):
      | Aileron: aileron, inboard elevon, outboard elevon
      | Elevator: aft-flap, inboard elvon, outboard elevon
      | Rudder: pylon rudder, winglet rudder
  Aileron : Inport
  Elevator : Inport  Port=2
  Rudder : Inport  Port=3
  Throttle : Inport  Port=4
  Nosegear : Inport  Port=5
  Brake : Inport  Port=6
  Flap : Inport  Port=7
  Feedback Bus : Inport  Port=8
  Bus Creator : BusCreator  Inputs=10
  Bus Creator1 : BusCreator  Inputs=4
  Bus Creator2 : BusCreator  Inputs=2
  Bus Creator3 : BusCreator  Inputs=2
  Bus Creator4 : BusCreator  Inputs=2
  Constant : Constant  Value=FTV
  Constant1 : Constant  Value=0
  FlapLhIBCmdDeg : Constant  Commented=on  Value=Trim_REFSI_FD_IN_nmodeFlapLhIBCmd_Deg
  FlapLhIBCmdDeg1 : Constant  Value=Trim_REFSI_FD_IN_nmodeFlapLhIBCmd_Deg
  Gain{1..5,8..9,12..17} (13 alike) : Gain
  Gain10 : Gain  Gain=-1
  Gain11 : Gain  Gain=-1
  Signal Specification{,1..3} (4 alike) : SignalSpecification  Dimensions=[1 1]  SampleTime=dt
  SlatLhPosnDeg : Constant  Value=Trim_REFSI_FD_IN_nmodeSlatLhCmd_Deg
  StabCmdDeg : Constant  Value=Trim_REFSI_FD_IN_nmodeStabCmd
  Surface Mixing Function : MATLAB Function  TreatAsAtomicUnit=on
  Switch : Switch  Criteria=u2 > Threshold  Threshold=2
  Terminator : Terminator
  Variant Model : $bdroot/Control Allocation/M2 Flap-to-Drag /Variant Model  SystemSampleTime=-1  Latency=0  AutoFrameSizeCalculation=off
  nmodeTlaLhCmdDeg3 : Constant  Value=Trim_REFSI_FD_IN_nmodeSplrLhOutbdCmd_Deg
  "Aileron_Deg " : Outport
  "InboardElevon_Deg " : Outport  Port=2
  OutboardElevon_Deg : Outport  Port=3
  "U-TailElevator_Deg " : Outport  Port=4
  Aft-Flap_Deg : Outport  Port=5
  PylonRudder_Deg : Outport  Port=6
  WingletRudder_Deg : Outport  Port=7
  U-tailRudder_Deg : Outport  Port=8
  "Throttle_Pct " : Outport  Port=9
  Nosegear_Deg : Outport  Port=10
  Brake (0-1) : Outport  Port=11
  Flaps_Deg : Outport  Port=12
  Slats_Deg : Outport  Port=13
  Spoilers_Deg : Outport  Port=14
  Stabilizer_Deg : Outport  Port=15
  tag scope: Sim_Surface=global
  wires:
  Gain4/1 -> Switch/1
  Constant1/1 -> Switch/3
  Switch/1 -> WingletRudder_Deg/1  "WingletRudder_Deg"
  Constant/1 -> Switch/2
  Signal Specification1/1 -> Surface Mixing Function/2(Pic_ElevatorCmd)
  Signal Specification2/1 -> Surface Mixing Function/3(Pic_RudderCmd)
  Signal Specification/1 -> Surface Mixing Function/1(Pic_AileronCmd)
  Gain5/1 -> U-tailRudder_Deg/1  "UtailRudder_Deg"
  Gain3/1 -> PylonRudder_Deg/1  "PylonRudder_Deg"
  Gain2/1 -> Aft-Flap_Deg/1  "AftFlap_deg"
  Gain1/1 -> "U-TailElevator_Deg "/1  "UtailElevator_Deg"
  Surface Mixing Function/5(PrtInbElevonCmd) -> Gain12/1
  Surface Mixing Function/6(StbdInbdElevonCmd) -> Gain13/1
  Surface Mixing Function/7(PrtOutElevonCmd) -> Gain14/1
  Surface Mixing Function/8(StbdOutdElevonCmd) -> Gain15/1
  Surface Mixing Function/9(ElevatorUtailCmd) -> Gain1/1
  Surface Mixing Function/10(AftFlapCmd) -> Gain2/1
  Surface Mixing Function/11(PylonRudderCmd) -> Gain3/1
  Surface Mixing Function/12(WingletRudderCmd) -> Gain4/1
  Surface Mixing Function/13(UTailRudderCmd) -> Gain5/1
  Surface Mixing Function/4(StbdAileronLowerCmd) -> Gain11/1
  Surface Mixing Function/3(StbdAileronUpperCmd) -> Gain10/1
  Surface Mixing Function/2(PrtAileronLowerCmd) -> Gain9/1
  Surface Mixing Function/1(PrtAileronUpperCmd) -> Gain8/1
  Flap/1 -> Signal Specification3/1, Bus Creator/7  "Sim_FlapsCmd"
  StabCmdDeg/1 -> Stabilizer_Deg/1, Bus Creator/10  "Sim_StabilizerCmd"
  Feedback Bus/1 -> Terminator/1
  nmodeTlaLhCmdDeg3/1 -> Spoilers_Deg/1, Bus Creator/9  "Sim_SpoilersCmd"
  SlatLhPosnDeg/1 -> Slats_Deg/1, Bus Creator/8  "Sim_SlatsCmd"
  Gain17/1 -> Bus Creator4/2  "StbdThrottleCmd_Pct"
  Bus Creator4/1 -> "Throttle_Pct "/1
  Gain16/1 -> Bus Creator4/1  "PrtThrottleCmd_Pct"
  Gain15/1 -> Bus Creator3/2  "StbdOutElevonCmd_Deg"
  Gain14/1 -> Bus Creator3/1  "PrtOutElevonCmd_Deg"
  Gain13/1 -> Bus Creator2/2  "StbdInbElevonCmd_Deg"
  Gain12/1 -> Bus Creator2/1  "PrtInbElevonCmd_Deg"
  Gain11/1 -> Bus Creator1/4  "StbdAileronLowerCmd_Deg"
  Gain10/1 -> Bus Creator1/3  "StbdAileronUpperCmd_Deg"
  Gain9/1 -> Bus Creator1/2  "PrtAileronLowerCmd_Deg"
  Gain8/1 -> Bus Creator1/1  "PrtAileronUpperCmd_Deg"
  Bus Creator3/1 -> OutboardElevon_Deg/1
  Bus Creator2/1 -> "InboardElevon_Deg "/1
  Bus Creator1/1 -> "Aileron_Deg "/1
  Variant Model/1 -> Gain16/1, Gain17/1  "Sim_ThrottleCmd"
  Throttle/1 -> Variant Model/1, Bus Creator/4  "Sim_ThrottleCmd"
  Bus Creator/1 -> [Sim_Surface]
  Brake/1 -> Bus Creator/6, Brake (0-1)/1  "Sim_BrakeCmd"
  Nosegear/1 -> Nosegear_Deg/1, Bus Creator/5  "Sim_NosegearCmd"
  Rudder/1 -> Signal Specification2/1, Bus Creator/3  "Sim_RudderCmd"
  Aileron/1 -> Signal Specification/1, Bus Creator/1  "Sim_AileronCmd"
  Elevator/1 -> Signal Specification1/1, Bus Creator/2  "Sim_ElevatorCmd"
  FlapLhIBCmdDeg1/1 -> Flaps_Deg/1  "REFSI_FD_IN_nmodeFlapLhOBPosn_Deg"
  Signal Specification3/1 -> Surface Mixing Function/4(Pic_FlapCmd)

== system Lib_Piccolo/Control Allocation/M2_OLD ==
  note: For 16.5% U-tail:
      | Aileron: aileron, inboard elevon, outboard elevon
      | Elevator: aft-flap, U-tail elevator,
      | Rudder: pylon rudder, winglet rudder, U-tail rudder
      |
      | For 16.5% Tailless (w/o U-tail elevator and U-tail rudder):
      | Aileron: aileron, inboard elevon, outboard elevon
      | Elevator: aft-flap, inboard elvon, outboard elevon
      | Rudder: pylon rudder, winglet rudder
  Aileron : Inport
  Elevator : Inport  Port=2
  Rudder : Inport  Port=3
  Throttle : Inport  Port=4
  Nosegear : Inport  Port=5
  Brake : Inport  Port=6
  Feedback Bus : Inport  Port=7
  Bus Creator : BusCreator  Inputs=6
  Bus Creator1 : BusCreator  Inputs=4
  Bus Creator2 : BusCreator  Inputs=2
  Bus Creator3 : BusCreator  Inputs=2
  Bus Creator4 : BusCreator  Inputs=2
  FlapLhIBCmdDeg : Constant  Value=Trim_REFSI_FD_IN_nmodeFlapLhIBCmd_Deg
  Gain{,1..9,12,14,16..18} (15 alike) : Gain
  Gain{10..11,13,15} (4 alike) : Gain  Gain=-1
  SlatLhPosnDeg : Constant  Value=Trim_REFSI_FD_IN_nmodeSlatLhCmd_Deg
  StabCmdDeg : Constant  Value=Trim_REFSI_FD_IN_nmodeStabCmd
  Terminator : Terminator
  Variant Model : Subsystem  Variant=on
  nmodeTlaLhCmdDeg3 : Constant  Value=Trim_REFSI_FD_IN_nmodeSplrLhOutbdCmd_Deg
  "Aileron_Deg " : Outport
  "InboardElevon_Deg " : Outport  Port=2
  OutboardElevon_Deg : Outport  Port=3
  "U-TailElevator_Deg " : Outport  Port=4
  Aft-Flap_Deg : Outport  Port=5
  PylonRudder_Deg : Outport  Port=6
  WingletRudder_Deg : Outport  Port=7
  U-tailRudder_Deg : Outport  Port=8
  "Throttle_Pct " : Outport  Port=9
  Nosegear_Deg : Outport  Port=10
  Brake (0-1) : Outport  Port=11
  Flaps_Deg : Outport  Port=12
  Slats_Deg : Outport  Port=13
  Spoilers_Deg : Outport  Port=14
  Stabilizer_Deg : Outport  Port=15
  tag scope: Sim_Surface=global
  wires:
  Elevator/1 -> Bus Creator/2, Gain1/1, Gain/1  "Sim_ElevatorCmd"
  Gain/1 -> "U-TailElevator_Deg "/1
  Aileron/1 -> Bus Creator/1, Gain2/1, Gain3/1, Gain4/1  "Sim_AileronCmd"
  Gain2/1 -> Gain8/1, Gain9/1, Gain10/1, Gain11/1
  Gain4/1 -> Gain14/1, Gain15/1
  Gain7/1 -> U-tailRudder_Deg/1
  Gain6/1 -> WingletRudder_Deg/1
  Gain5/1 -> PylonRudder_Deg/1
  Rudder/1 -> Bus Creator/3, Gain7/1, Gain6/1, Gain5/1  "Sim_RudderCmd"
  Gain1/1 -> Aft-Flap_Deg/1
  Nosegear/1 -> Bus Creator/5, Nosegear_Deg/1  "Sim_NosegearCmd"
  Brake/1 -> Brake (0-1)/1, Bus Creator/6  "Sim_BrakeCmd"
  Bus Creator/1 -> [Sim_Surface]
  Throttle/1 -> Bus Creator/4, Variant Model/1(Sim_ThrottleCmd)  "Sim_ThrottleCmd"
  Variant Model/1(ThrottleCmdOut) -> Gain18/1  "Sim_ThrottleCmd"
  Bus Creator1/1 -> "Aileron_Deg "/1
  Gain3/1 -> Gain12/1, Gain13/1
  Bus Creator2/1 -> "InboardElevon_Deg "/1
  Bus Creator3/1 -> OutboardElevon_Deg/1
  Gain8/1 -> Bus Creator1/1  "PrtAileronUpperCmd_Deg"
  Gain9/1 -> Bus Creator1/2  "PrtAileronLowerCmd_Deg"
  Gain10/1 -> Bus Creator1/3  "StbdAileronUpperCmd_Deg"
  Gain11/1 -> Bus Creator1/4  "StbdAileronLowerCmd_Deg"
  Gain12/1 -> Bus Creator2/1  "PrtInbElevonCmd_Deg"
  Gain13/1 -> Bus Creator2/2  "StbdInbElevonCmd_Deg"
  Gain14/1 -> Bus Creator3/1  "PrtOutElevonCmd_Deg"
  Gain15/1 -> Bus Creator3/2  "StbdOutElevonCmd_Deg"
  Gain16/1 -> Bus Creator4/1  "PrtThrottleCmd_Pct"
  Bus Creator4/1 -> "Throttle_Pct "/1
  Gain17/1 -> Bus Creator4/2  "StbdThrottleCmd_Pct"
  Gain18/1 -> Gain17/1, Gain16/1
  SlatLhPosnDeg/1 -> Slats_Deg/1  "REFSI_FD_IN_nmodeSlatLhCmd_Deg"
  nmodeTlaLhCmdDeg3/1 -> Spoilers_Deg/1  "REFSI_FD_IN_nmodeSplrLhOutbdCmd_Deg"
  Feedback Bus/1 -> Terminator/1
  StabCmdDeg/1 -> Stabilizer_Deg/1  "REFSI_FD_IN_nmodeStabCmd"
  FlapLhIBCmdDeg/1 -> Flaps_Deg/1  "REFSI_FD_IN_nmodeFlapLhOBPosn_Deg"
